simulink model "ts_b04_grid_PASS"  (R2024b)
settings: Solver=FixedStepDiscrete  StartTime=0.0  StopTime=12  FixedStep=Ts  RelTol=1e-4
PreLoadFcn:
  | Ts=50e-6;
undefined symbols (not defined in the file): D1, Delta, DiscIntNeverNeededParam
libraries: simulink x22, spsSecondOrderFilterLib x14, spsabctodq0Lib x7, spsThreePhaseVIMeasurementLib x7, spsThreePhaseSeriesRLCLoadLib x5, spsPowerPLLDrivenPositiveSequenceLib x4, spsStairGeneratorLib x4, spsThreePhaseTransformerTwoWindingsLib x3, spsDCVoltageSourceLib x3, spsThreePhaseSeriesRLCBranchLib x3, spsPWMGeneratorPulseAveragingLib x3, spsTwoLevelConverterLib x3
(part 2 of 3)

== system ts_b04_grid_PASS/Microgrid Supervisory Control/PI regulator with anti-windup q ==
  note: Anti-windup mechanism: Method of conditionnal integration
      |
      | The integration is suspended if saturation occurs and the
      | control error is of the same sign as the control signal.
      |
      | [1] L.Rundqwist, "Anti-Reset Windup for PID Controllers," Ph.D. Thesis TRFT-1033,
      | Departement of Automatic Control, Lund Institute of Technology, Lund, Sweeden, 1991.
  Error : Inport  SampleTime=Ts
  Reset : Inport  Port=2  SampleTime=Ts
  Compare To Zero : simulink/Logic and Bit Operations/Compare To Zero  relop=>  OutDataTypeStr=uint8  ZeroCross=off
  Compare To Zero1 : simulink/Logic and Bit Operations/Compare To Zero  relop=<  OutDataTypeStr=uint8  ZeroCross=off
  Constant : Constant  Value=0
  Constant1 : Constant  Value=UpperLimit
  Constant3 : Constant  Value=LowerLimit
  Discrete-Time Integrator : DiscreteIntegrator  IntegratorMethod=Integration: Trapezoidal  ExternalReset=level  InitialCondition=Init  SampleTime=Ts  LimitOutput=on  UpperSaturationLimit=UpperLimit  LowerSaturationLimit=LowerLimit  ShowStatePort=on  ICPrevOutput=DiscIntNeverNeededParam  ICPrevScaledInput=DiscIntNeverNeededParam
  Kp4 : Gain  Gain=Kp  SaturateOnIntegerOverflow=on  SampleTime=Ts  OutDataTypeStr=Inherit: Same as input  ParamDataTypeStr=Inherit: Same as input
  Kp5 : Gain  Gain=Ki  SaturateOnIntegerOverflow=on  SampleTime=Ts  OutDataTypeStr=Inherit: Same as input  ParamDataTypeStr=Inherit: Same as input
  Logical Operator : Logic  AllPortsSameDT=off  OutDataTypeStr=boolean
  Logical Operator1 : Logic  AllPortsSameDT=off  OutDataTypeStr=boolean
  Logical Operator2 : Logic  Operator=OR  AllPortsSameDT=off  OutDataTypeStr=boolean
  Relational Operator : RelationalOperator  OutDataTypeStr=boolean  InputSameDT=off
  Relational Operator1 : RelationalOperator  Operator=<=  OutDataTypeStr=boolean  InputSameDT=off
  Saturation2 : Saturate  UpperLimit=UpperLimit  LowerLimit=LowerLimit  SampleTime=Ts
  Sum1 : Sum  InputSameDT=on  SaturateOnIntegerOverflow=on  SampleTime=Ts  OutDataTypeStr=Inherit: Same as first input
  Sum6 : Sum  InputSameDT=on  SaturateOnIntegerOverflow=on  SampleTime=Ts  OutDataTypeStr=Inherit: Same as first input
  Switch : Switch  Criteria=u2 > Threshold  SaturateOnIntegerOverflow=off  InputSameDT=off
  Zero-Order Hold : ZeroOrderHold  SampleTime=Ts
  Out : Outport  SampleTime=Ts  InitialOutput=0  VectorParamsAs1DForOutWhenUnconnected=off
  wires:
  Reset/1 -> Discrete-Time Integrator/2
  Constant/1 -> Switch/1
  Zero-Order Hold/1 -> Sum1/2, Sum6/1
  Discrete-Time Integrator/State -> Sum1/1
  Sum1/1 -> Relational Operator1/1, Relational Operator/1
  Logical Operator2/1 -> Switch/2
  Relational Operator/1 -> Logical Operator/1  "UpperLimit_is_Reached"
  Relational Operator1/1 -> Logical Operator1/1  "LowerLimit_Is_Reached"
  Constant1/1 -> Relational Operator/2
  Constant3/1 -> Relational Operator1/2
  Compare To Zero/1 -> Logical Operator/2  "Error_is_positive"
  Logical Operator/1 -> Logical Operator2/1
  Logical Operator1/1 -> Logical Operator2/2
  Compare To Zero1/1 -> Logical Operator1/2  "Error_is_negative"
  Error/1 -> Compare To Zero1/1, Compare To Zero/1, Kp4/1, Kp5/1
  Sum6/1 -> Saturation2/1
  Kp4/1 -> Zero-Order Hold/1
  Discrete-Time Integrator/1 -> Sum6/2
  Saturation2/1 -> Out/1
  Switch/1 -> Discrete-Time Integrator/1
  Kp5/1 -> Switch/3

== system ts_b04_grid_PASS/Microgrid Supervisory Control/PI regulator with anti-windup q1 ==
  note: Anti-windup mechanism: Method of conditionnal integration
      |
      | The integration is suspended if saturation occurs and the
      | control error is of the same sign as the control signal.
      |
      | [1] L.Rundqwist, "Anti-Reset Windup for PID Controllers," Ph.D. Thesis TRFT-1033,
      | Departement of Automatic Control, Lund Institute of Technology, Lund, Sweeden, 1991.
  Error : Inport  SampleTime=Ts
  Reset : Inport  Port=2  SampleTime=Ts
  Compare To Zero : simulink/Logic and Bit Operations/Compare To Zero  relop=>  OutDataTypeStr=uint8  ZeroCross=off
  Compare To Zero1 : simulink/Logic and Bit Operations/Compare To Zero  relop=<  OutDataTypeStr=uint8  ZeroCross=off
  Constant : Constant  Value=0
  Constant1 : Constant  Value=UpperLimit
  Constant3 : Constant  Value=LowerLimit
  Discrete-Time Integrator : DiscreteIntegrator  IntegratorMethod=Integration: Trapezoidal  ExternalReset=level  InitialCondition=Init  SampleTime=Ts  LimitOutput=on  UpperSaturationLimit=UpperLimit  LowerSaturationLimit=LowerLimit  ShowStatePort=on  ICPrevOutput=DiscIntNeverNeededParam  ICPrevScaledInput=DiscIntNeverNeededParam
  Kp4 : Gain  Gain=Kp  SaturateOnIntegerOverflow=on  SampleTime=Ts  OutDataTypeStr=Inherit: Same as input  ParamDataTypeStr=Inherit: Same as input
  Kp5 : Gain  Gain=Ki  SaturateOnIntegerOverflow=on  SampleTime=Ts  OutDataTypeStr=Inherit: Same as input  ParamDataTypeStr=Inherit: Same as input
  Logical Operator : Logic  AllPortsSameDT=off  OutDataTypeStr=boolean
  Logical Operator1 : Logic  AllPortsSameDT=off  OutDataTypeStr=boolean
  Logical Operator2 : Logic  Operator=OR  AllPortsSameDT=off  OutDataTypeStr=boolean
  Relational Operator : RelationalOperator  OutDataTypeStr=boolean  InputSameDT=off
  Relational Operator1 : RelationalOperator  Operator=<=  OutDataTypeStr=boolean  InputSameDT=off
  Saturation2 : Saturate  UpperLimit=UpperLimit  LowerLimit=LowerLimit  SampleTime=Ts
  Sum1 : Sum  InputSameDT=on  SaturateOnIntegerOverflow=on  SampleTime=Ts  OutDataTypeStr=Inherit: Same as first input
  Sum6 : Sum  InputSameDT=on  SaturateOnIntegerOverflow=on  SampleTime=Ts  OutDataTypeStr=Inherit: Same as first input
  Switch : Switch  Criteria=u2 > Threshold  SaturateOnIntegerOverflow=off  InputSameDT=off
  Zero-Order Hold : ZeroOrderHold  SampleTime=Ts
  Out : Outport  SampleTime=Ts  InitialOutput=0  VectorParamsAs1DForOutWhenUnconnected=off
  wires:
  Kp5/1 -> Switch/3
  Switch/1 -> Discrete-Time Integrator/1
  Saturation2/1 -> Out/1
  Discrete-Time Integrator/1 -> Sum6/2
  Kp4/1 -> Zero-Order Hold/1
  Sum6/1 -> Saturation2/1
  Error/1 -> Kp5/1, Kp4/1, Compare To Zero/1, Compare To Zero1/1
  Compare To Zero1/1 -> Logical Operator1/2  "Error_is_negative"
  Logical Operator1/1 -> Logical Operator2/2
  Logical Operator/1 -> Logical Operator2/1
  Compare To Zero/1 -> Logical Operator/2  "Error_is_positive"
  Constant3/1 -> Relational Operator1/2
  Constant1/1 -> Relational Operator/2
  Relational Operator1/1 -> Logical Operator1/1  "LowerLimit_Is_Reached"
  Relational Operator/1 -> Logical Operator/1  "UpperLimit_is_Reached"
  Logical Operator2/1 -> Switch/2
  Sum1/1 -> Relational Operator/1, Relational Operator1/1
  Discrete-Time Integrator/State -> Sum1/1
  Zero-Order Hold/1 -> Sum6/1, Sum1/2
  Constant/1 -> Switch/1
  Reset/1 -> Discrete-Time Integrator/2

== system ts_b04_grid_PASS/Inverter 1 500 kW/Control System/Current Regulator ==
  note: For Ltot >> Rtot :
  note: (Vq_prim - Vq_conv) ~ = - Id * Ltot
  note: (Vd_prim - Vd_conv) ~= + Iq * Ltot
  note: Ltot = Lxfo + Lchoke
      | Rtot = Rxfo + Rchoke
  note: Id positive --> The converter generates active power ("Inverter mode") = Active Power P positive
  note: Iq positive --> The converter absorbs reactive power ("Inductive mode") = Reactive Power Q negative
  note: Sign Convention: Current going out of the converter = positive current
  note: Current Regulator
      | (with feedforward)
  note: Vq_meas + Id*L + Iq*R + deriv(Iq)*L/wbase= Vq_conv
  note: Vd_meas + Id*R - Iq*L + deriv(Id)*L/wbase= Vd_conv
  note: harmonic filter neglected
  VdVq_meas : Inport  PortDimensions=2
  IdIq_meas : Inport  Port=2  PortDimensions=2
  IdIq_ref : Inport  Port=3  PortDimensions=2
  Add1 : Sum  Inputs=++-
  Add2 : Sum
  Add3 : Sum  Inputs=+++
  Demux : Demux  Outputs=2
  Demux1 : Demux  Outputs=2
  Ltot_pu1 : Gain  Gain=Lff  SaturateOnIntegerOverflow=on  OutDataTypeStr=Inherit: Same as input  ParamDataTypeStr=Inherit: Same as input
  Ltot_pu2 : Gain  Gain=Lff  SaturateOnIntegerOverflow=on  OutDataTypeStr=Inherit: Same as input  ParamDataTypeStr=Inherit: Same as input
  Mux : Mux  Inputs=2
  PI regulator with anti-windup D : Subsystem  DialogController=POWERSYS.PowerSysDialog  mask(Discrete PI Controller){Kp=Kp_Ireg, Ki=Ki_Ireg, Par_Limits=Limits_Ireg, Init=0, Ts=Ts}
      mask prompts: Kp "Proportional gain (Kp):"; Ki "Integral gain (Ki):"; Par_Limits "Output limits: [ Upper   Lower ]"; Init "Output initial value:"; Ts "Sample time:"
      mask help: This block implements a discrete PI controller.
      mask init:
      | UpperLimit=Par_Limits(1);
      | LowerLimit=Par_Limits(2);
      | power_initmask();
      mask Help: This block is part of a subset of blocks in the Extras library that does not have documentation associated with it, other than the block mask description.
      mask Display: disp('PI');
  Rtot_pu1 : Gain  Gain=Rff  SaturateOnIntegerOverflow=on  OutDataTypeStr=Inherit: Same as input  ParamDataTypeStr=Inherit: Same as input
  Rtot_pu5 : Gain  Gain=Rff  SaturateOnIntegerOverflow=on  OutDataTypeStr=Inherit: Same as input  ParamDataTypeStr=Inherit: Same as input
  Saturation : Saturate  UpperLimit=Limits_Ireg(1)  LowerLimit=Limits_Ireg(2)
  Sum : Sum  Inputs=|-+
  VdVq_conv : Outport  VectorParamsAs1DForOutWhenUnconnected=off
  PIdq : Outport  Port=2  VectorParamsAs1DForOutWhenUnconnected=off
  wires:
  Add3/1 -> Mux/2
  Demux/2 -> Add3/1
  Add1/1 -> Mux/1  "Feedforward"
  Ltot_pu2/1 -> Add3/3
  Rtot_pu5/1 -> Add3/2
  Demux1/2 -> Rtot_pu5/1, Ltot_pu1/1
  Ltot_pu1/1 -> Add1/3
  Demux1/1 -> Ltot_pu2/1, Rtot_pu1/1
  Rtot_pu1/1 -> Add1/2
  Demux/1 -> Add1/1
  VdVq_meas/1 -> Demux/1
  Saturation/1 -> VdVq_conv/1
  Add2/1 -> Saturation/1
  IdIq_meas/1 -> Sum/1
  IdIq_ref/1 -> Demux1/1, Sum/2
  Sum/1 -> PI regulator with anti-windup D/1(Error)
  PI regulator with anti-windup D/1(Out) -> Add2/1, PIdq/1  "PI"
  Mux/1 -> Add2/2

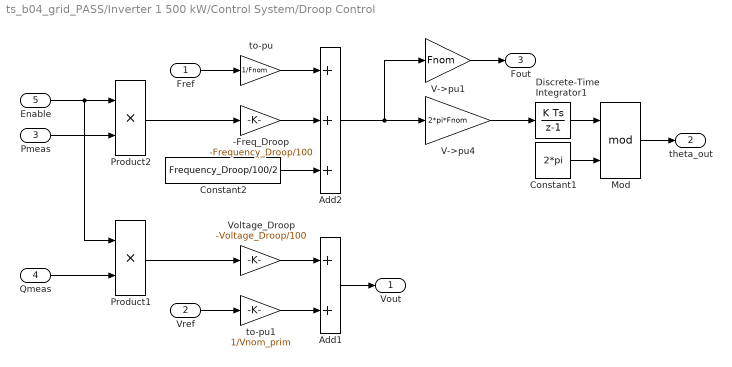
== system ts_b04_grid_PASS/Inverter 1 500 kW/Control System/Droop Control ==
  Fref : Inport  PortDimensions=1
  Vref : Inport  Port=2  PortDimensions=1
  Pmeas : Inport  Port=3
  Qmeas : Inport  Port=4
  Enable : Inport  Port=5
  -Freq_Droop : Gain  Gain=-Frequency_Droop/100
  Add1 : Sum
  Add2 : Sum  Inputs=+++
  Constant1 : Constant  Value=2*pi
  Constant2 : Constant  Value=Frequency_Droop/100/2
  Discrete-Time Integrator1 : DiscreteIntegrator  SampleTime=Ts  ICPrevOutput=DiscIntNeverNeededParam  ICPrevScaledInput=DiscIntNeverNeededParam
  Mod : Math  Operator=mod
  Product1 : Product
  Product2 : Product
  V->pu1 : Gain  Gain=Fnom  SaturateOnIntegerOverflow=on  OutDataTypeStr=Inherit: Same as input  ParamDataTypeStr=Inherit: Same as input
  V->pu4 : Gain  Gain=2*pi*Fnom  SaturateOnIntegerOverflow=on  OutDataTypeStr=Inherit: Same as input  ParamDataTypeStr=Inherit: Same as input
  Voltage_Droop : Gain  Gain=-Voltage_Droop/100
  to-pu : Gain  Gain=1/Fnom
  to-pu1 : Gain  Gain=1/Vnom_prim
  Vout : Outport
  theta_out : Outport  Port=2
  Fout : Outport  Port=3
  wires:
  Constant1/1 -> Mod/2
  -Freq_Droop/1 -> Add2/2
  Discrete-Time Integrator1/1 -> Mod/1
  Add2/1 -> V->pu4/1, V->pu1/1
  Enable/1 -> Product1/1, Product2/1
  Pmeas/1 -> Product2/2
  to-pu/1 -> Add2/1
  V->pu4/1 -> Discrete-Time Integrator1/1
  Fref/1 -> to-pu/1
  Vref/1 -> to-pu1/1
  to-pu1/1 -> Add1/2
  Add1/1 -> Vout/1
  Mod/1 -> theta_out/1
  Voltage_Droop/1 -> Add1/1
  Qmeas/1 -> Product1/2
  Product2/1 -> -Freq_Droop/1
  Product1/1 -> Voltage_Droop/1
  Constant2/1 -> Add2/3
  V->pu1/1 -> Fout/1

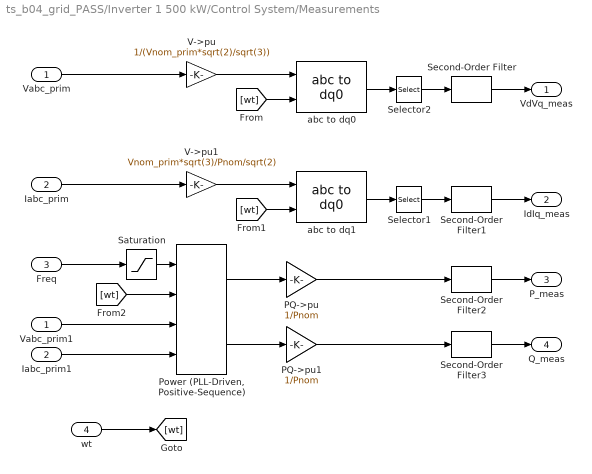
== system ts_b04_grid_PASS/Inverter 1 500 kW/Control System/Measurements ==
  Vabc_prim : Inport
  Iabc_prim : Inport  Port=2
  Freq : Inport  Port=3
  wt : Inport  Port=4
  Iabc_prim1 : InportShadow  Port=2
  PQ->pu : Gain  Gain=1/Pnom  SaturateOnIntegerOverflow=on  OutDataTypeStr=Inherit: Same as input  ParamDataTypeStr=Inherit: Same as input
  PQ->pu1 : Gain  Gain=1/Pnom  SaturateOnIntegerOverflow=on  OutDataTypeStr=Inherit: Same as input  ParamDataTypeStr=Inherit: Same as input
  "Power (PLL-Driven, Positive-Sequence)" : spsPowerPLLDrivenPositiveSequenceLib/Power (PLL-Driven, Positive-Sequence)  Finit=50  Fmin=45  Vinit=[1, 0]  Iinit=[1, 0]  Ts=Ts
  Saturation : Saturate  UpperLimit=55  LowerLimit=45
  Second-Order Filter{,1..3} (4 alike) : spsSecondOrderFilterLib/Second-Order Filter  FilterType=Lowpass  Fo=fn_Filter  Zeta=1  Ts=Ts  Initialize=off  Vac_Init=[0, 0, 50]  Vdc_Init=0  PlotResponse=off  FreqRange=[0, 500, 1]
  Selector1 : Selector  InputPortWidth=3  IndexOptions=Index vector (dialog)  Indices=[1 2]  OutputSizes=1
  Selector2 : Selector  InputPortWidth=3  IndexOptions=Index vector (dialog)  Indices=[1 2]  OutputSizes=1
  V->pu : Gain  Gain=1/(Vnom_prim*sqrt(2)/sqrt(3))  SaturateOnIntegerOverflow=on  OutDataTypeStr=Inherit: Same as input  ParamDataTypeStr=Inherit: Same as input
  V->pu1 : Gain  Gain=Vnom_prim*sqrt(3)/Pnom/sqrt(2)  SaturateOnIntegerOverflow=on  OutDataTypeStr=Inherit: Same as input  ParamDataTypeStr=Inherit: Same as input
  Vabc_prim1 : InportShadow
  abc to dq0 : spsabctodq0Lib/abc to dq0  Alignment=90 degrees behind phase A axis
  abc to dq1 : spsabctodq0Lib/abc to dq0  Alignment=90 degrees behind phase A axis
  VdVq_meas : Outport  VectorParamsAs1DForOutWhenUnconnected=off
  IdIq_meas : Outport  Port=2  VectorParamsAs1DForOutWhenUnconnected=off
  P_meas : Outport  Port=3  VectorParamsAs1DForOutWhenUnconnected=off
  Q_meas : Outport  Port=4  VectorParamsAs1DForOutWhenUnconnected=off
  wires:
  Iabc_prim1/1 -> "Power (PLL-Driven, Positive-Sequence)"/4
  Vabc_prim1/1 -> "Power (PLL-Driven, Positive-Sequence)"/3
  abc to dq0/1 -> Selector2/1
  Iabc_prim/1 -> V->pu1/1
  Vabc_prim/1 -> V->pu/1
  abc to dq1/1 -> Selector1/1
  V->pu/1 -> abc to dq0/1
  V->pu1/1 -> abc to dq1/1
  Freq/1 -> Saturation/1
  Selector2/1 -> Second-Order Filter/1
  Selector1/1 -> Second-Order Filter1/1
  Second-Order Filter/1 -> VdVq_meas/1
  Second-Order Filter1/1 -> IdIq_meas/1
  [wt] -> abc to dq0/2
  [wt] -> abc to dq1/2
  [wt] -> "Power (PLL-Driven, Positive-Sequence)"/2
  "Power (PLL-Driven, Positive-Sequence)"/1 -> PQ->pu/1
  Second-Order Filter2/1 -> P_meas/1
  PQ->pu1/1 -> Second-Order Filter3/1
  Second-Order Filter3/1 -> Q_meas/1
  PQ->pu/1 -> Second-Order Filter2/1
  "Power (PLL-Driven, Positive-Sequence)"/2 -> PQ->pu1/1
  wt/1 -> [wt]
  Saturation/1 -> "Power (PLL-Driven, Positive-Sequence)"/1

== system ts_b04_grid_PASS/Inverter 1 500 kW/Control System/Voltage Regulators ==
  note: Iqref limit set 0.5 pu
  Vq : Inport  PortDimensions=1
  Vq_ref : Inport  Port=2  PortDimensions=1
  On : Inport  Port=3  PortDimensions=1
  Vd : Inport  Port=4  PortDimensions=1
  Vd_ref : Inport  Port=5  PortDimensions=1
  Constant1 : Constant  Value=0
  Constant2 : Constant
  Mux : Mux  Inputs=2
  PI regulator with anti-windup 1 : Subsystem  DialogController=POWERSYS.PowerSysDialog  mask(Discrete PI Controller){Kp=Kp_Vreg, Ki=Ki_Vreg, Par_Limits=[0.5, -0.5], Init=0, Ts=Ts}
      mask prompts: Kp "Proportional gain (Kp):"; Ki "Integral gain (Ki):"; Par_Limits "Output limits: [ Upper   Lower ]"; Init "Output initial value:"; Ts "Sample time:"
      mask help: This block implements a discrete PI controller.
      mask init:
      | UpperLimit=Par_Limits(1);
      | LowerLimit=Par_Limits(2);
      | power_initmask();
      mask Help: This block is part of a subset of blocks in the Extras library that does not have documentation associated with it, other than the block mask description.
      mask Display: disp('PI');
  PI regulator with anti-windup 2 : Subsystem  DialogController=POWERSYS.PowerSysDialog  mask(Discrete PI Controller){Kp=Kp_Vreg, Ki=Ki_Vreg, Par_Limits=Limits_Vreg, Init=0, Ts=Ts}
      mask prompts: Kp "Proportional gain (Kp):"; Ki "Integral gain (Ki):"; Par_Limits "Output limits: [ Upper   Lower ]"; Init "Output initial value:"; Ts "Sample time:"
      mask help: This block implements a discrete PI controller.
      mask init:
      | UpperLimit=Par_Limits(1);
      | LowerLimit=Par_Limits(2);
      | power_initmask();
      mask Help: This block is part of a subset of blocks in the Extras library that does not have documentation associated with it, other than the block mask description.
      mask Display: disp('PI');
  Sum : Sum  Inputs=|+-
  Sum1 : Sum  Inputs=|+-
  Switch : Switch  Criteria=u2 ~= 0  SaturateOnIntegerOverflow=off  InputSameDT=off
  IdIq_ref : Outport  InitialOutput=0  VectorParamsAs1DForOutWhenUnconnected=off
  wires:
  Constant1/1 -> Switch/1
  On/1 -> Switch/2
  Switch/1 -> PI regulator with anti-windup 2/2(Reset), PI regulator with anti-windup 1/2(Reset)
  Constant2/1 -> Switch/3
  Vq_ref/1 -> Sum/1
  Vq/1 -> Sum/2
  Sum/1 -> PI regulator with anti-windup 1/1(Error)
  Sum1/1 -> PI regulator with anti-windup 2/1(Error)
  Vd/1 -> Sum1/1
  Vd_ref/1 -> Sum1/2
  PI regulator with anti-windup 2/1(Out) -> Mux/2
  Mux/1 -> IdIq_ref/1
  PI regulator with anti-windup 1/1(Out) -> Mux/1

== system ts_b04_grid_PASS/Inverter 1 500 kW/Control System/Vref Generation ==
  note: (Correction for delai of Ts)
  note: (Correction for transformer
      |  D1 connection)
  wt : Inport
  VdVq_conv : Inport  Port=2
  Vdc_meas : Inport  Port=3
  Add1 : Sum  Inputs=++++
  Add2 : Sum
  Complex to Magnitude-Angle : ComplexToMagnitudeAngle
  Constant : Constant  Value=-pi/6
  Constant2 : Constant  Value="[ 0  -2*pi/3  2*pi/3  ]"
  Constant3 : Constant  Value=Vnom_sec*sqrt(2)/sqrt(3)
  Constant4 : Constant  Value=Ts*Fnom*(2*pi)
  Demux1 : Demux  Outputs=2
  Gain1 : Gain  Gain=1/2
  Product : Product  Inputs=*/  RndMeth=Zero
  Product1 : Product  Inputs=*/  RndMeth=Zero
  Product2 : Product  Inputs=**  RndMeth=Zero
  Real-Imag to Complex : RealImagToComplex
  Saturation : Saturate  UpperLimit=1  LowerLimit=0
  Trigonometric Function : Trigonometry
  Vref : Outport  VectorParamsAs1DForOutWhenUnconnected=off
  ModIndex : Outport  Port=2  VectorParamsAs1DForOutWhenUnconnected=off
  wires:
  Constant4/1 -> Add1/4
  wt/1 -> Add1/1
  Product2/1 -> Vref/1
  Trigonometric Function/1 -> Product2/2
  Saturation/1 -> ModIndex/1, Product2/1
  Add2/1 -> Trigonometric Function/1
  Add1/1 -> Add2/2
  Complex to Magnitude-Angle/2 -> Add2/1
  Product/1 -> Product1/2
  Constant3/1 -> Product/2
  Constant/1 -> Add1/3
  Constant2/1 -> Add1/2
  Demux1/2 -> Real-Imag to Complex/2
  Demux1/1 -> Real-Imag to Complex/1
  Real-Imag to Complex/1 -> Complex to Magnitude-Angle/1
  Gain1/1 -> Product/1
  Product1/1 -> Demux1/1
  VdVq_conv/1 -> Product1/1
  Vdc_meas/1 -> Gain1/1
  Complex to Magnitude-Angle/1 -> Saturation/1

== system ts_b04_grid_PASS/Inverter 2 300 kW/Control System/Current Regulator ==
  note: For Ltot >> Rtot :
  note: (Vq_prim - Vq_conv) ~ = - Id * Ltot
  note: (Vd_prim - Vd_conv) ~= + Iq * Ltot
  note: Ltot = Lxfo + Lchoke
      | Rtot = Rxfo + Rchoke
  note: Id positive --> The converter generates active power ("Inverter mode") = Active Power P positive
  note: Iq positive --> The converter absorbs reactive power ("Inductive mode") = Reactive Power Q negative
  note: Sign Convention: Current going out of the converter = positive current
  note: Current Regulator
      | (with feedforward)
  note: Vq_meas + Id*L + Iq*R + deriv(Iq)*L/wbase= Vq_conv
  note: Vd_meas + Id*R - Iq*L + deriv(Id)*L/wbase= Vd_conv
  note: harmonic filter neglected
  VdVq_meas : Inport  PortDimensions=2
  IdIq_meas : Inport  Port=2  PortDimensions=2
  IdIq_ref : Inport  Port=3  PortDimensions=2
  Add1 : Sum  Inputs=++-
  Add2 : Sum
  Add3 : Sum  Inputs=+++
  Demux : Demux  Outputs=2
  Demux1 : Demux  Outputs=2
  Ltot_pu1 : Gain  Gain=Lff  SaturateOnIntegerOverflow=on  OutDataTypeStr=Inherit: Same as input  ParamDataTypeStr=Inherit: Same as input
  Ltot_pu2 : Gain  Gain=Lff  SaturateOnIntegerOverflow=on  OutDataTypeStr=Inherit: Same as input  ParamDataTypeStr=Inherit: Same as input
  Mux : Mux  Inputs=2
  PI regulator with anti-windup D : Subsystem  DialogController=POWERSYS.PowerSysDialog  mask(Discrete PI Controller){Kp=Kp_Ireg, Ki=Ki_Ireg, Par_Limits=Limits_Ireg, Init=0, Ts=Ts}
      mask prompts: Kp "Proportional gain (Kp):"; Ki "Integral gain (Ki):"; Par_Limits "Output limits: [ Upper   Lower ]"; Init "Output initial value:"; Ts "Sample time:"
      mask help: This block implements a discrete PI controller.
      mask init:
      | UpperLimit=Par_Limits(1);
      | LowerLimit=Par_Limits(2);
      | power_initmask();
      mask Help: This block is part of a subset of blocks in the Extras library that does not have documentation associated with it, other than the block mask description.
      mask Display: disp('PI');
  Rtot_pu1 : Gain  Gain=Rff  SaturateOnIntegerOverflow=on  OutDataTypeStr=Inherit: Same as input  ParamDataTypeStr=Inherit: Same as input
  Rtot_pu5 : Gain  Gain=Rff  SaturateOnIntegerOverflow=on  OutDataTypeStr=Inherit: Same as input  ParamDataTypeStr=Inherit: Same as input
  Saturation : Saturate  UpperLimit=Limits_Ireg(1)  LowerLimit=Limits_Ireg(2)
  Sum : Sum  Inputs=|-+
  VdVq_conv : Outport  VectorParamsAs1DForOutWhenUnconnected=off
  PIdq : Outport  Port=2  VectorParamsAs1DForOutWhenUnconnected=off
  wires:
  Add3/1 -> Mux/2
  Demux/2 -> Add3/1
  Add1/1 -> Mux/1  "Feedforward"
  Ltot_pu2/1 -> Add3/3
  Rtot_pu5/1 -> Add3/2
  Demux1/2 -> Rtot_pu5/1, Ltot_pu1/1
  Ltot_pu1/1 -> Add1/3
  Demux1/1 -> Ltot_pu2/1, Rtot_pu1/1
  Rtot_pu1/1 -> Add1/2
  Demux/1 -> Add1/1
  VdVq_meas/1 -> Demux/1
  Saturation/1 -> VdVq_conv/1
  Add2/1 -> Saturation/1
  IdIq_meas/1 -> Sum/1
  IdIq_ref/1 -> Demux1/1, Sum/2
  Sum/1 -> PI regulator with anti-windup D/1(Error)
  PI regulator with anti-windup D/1(Out) -> Add2/1, PIdq/1  "PI"
  Mux/1 -> Add2/2

== system ts_b04_grid_PASS/Inverter 2 300 kW/Control System/Droop Control ==
  Fref : Inport  PortDimensions=1
  Vref : Inport  Port=2  PortDimensions=1
  Pmeas : Inport  Port=3
  Qmeas : Inport  Port=4
  Enable : Inport  Port=5
  -Freq_Droop : Gain  Gain=-Frequency_Droop/100
  Add1 : Sum
  Add2 : Sum  Inputs=+++
  Constant1 : Constant  Value=2*pi
  Constant2 : Constant  Value=Frequency_Droop/100/2
  Discrete-Time Integrator1 : DiscreteIntegrator  SampleTime=Ts  ICPrevOutput=DiscIntNeverNeededParam  ICPrevScaledInput=DiscIntNeverNeededParam
  Mod : Math  Operator=mod
  Product1 : Product
  Product2 : Product
  V->pu1 : Gain  Gain=Fnom  SaturateOnIntegerOverflow=on  OutDataTypeStr=Inherit: Same as input  ParamDataTypeStr=Inherit: Same as input
  V->pu4 : Gain  Gain=2*pi*Fnom  SaturateOnIntegerOverflow=on  OutDataTypeStr=Inherit: Same as input  ParamDataTypeStr=Inherit: Same as input
  Voltage_Droop : Gain  Gain=-Voltage_Droop/100
  to-pu : Gain  Gain=1/Fnom
  to-pu1 : Gain  Gain=1/Vnom_prim
  Vout : Outport
  theta_out : Outport  Port=2
  Fout : Outport  Port=3
  wires:
  Constant1/1 -> Mod/2
  -Freq_Droop/1 -> Add2/2
  Discrete-Time Integrator1/1 -> Mod/1
  Add2/1 -> V->pu4/1, V->pu1/1
  Enable/1 -> Product1/1, Product2/1
  Pmeas/1 -> Product2/2
  to-pu/1 -> Add2/1
  V->pu4/1 -> Discrete-Time Integrator1/1
  Fref/1 -> to-pu/1
  Vref/1 -> to-pu1/1
  to-pu1/1 -> Add1/2
  Add1/1 -> Vout/1
  Mod/1 -> theta_out/1
  Voltage_Droop/1 -> Add1/1
  Qmeas/1 -> Product1/2
  Product2/1 -> -Freq_Droop/1
  Product1/1 -> Voltage_Droop/1
  Constant2/1 -> Add2/3
  V->pu1/1 -> Fout/1

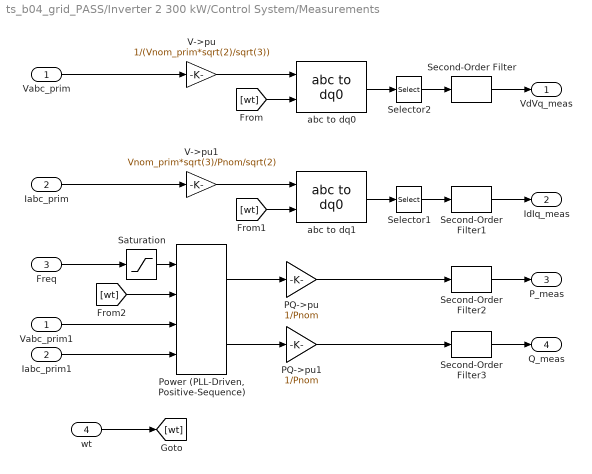
== system ts_b04_grid_PASS/Inverter 2 300 kW/Control System/Measurements ==
  Vabc_prim : Inport
  Iabc_prim : Inport  Port=2
  Freq : Inport  Port=3
  wt : Inport  Port=4
  Iabc_prim1 : InportShadow  Port=2
  PQ->pu : Gain  Gain=1/Pnom  SaturateOnIntegerOverflow=on  OutDataTypeStr=Inherit: Same as input  ParamDataTypeStr=Inherit: Same as input
  PQ->pu1 : Gain  Gain=1/Pnom  SaturateOnIntegerOverflow=on  OutDataTypeStr=Inherit: Same as input  ParamDataTypeStr=Inherit: Same as input
  "Power (PLL-Driven, Positive-Sequence)" : spsPowerPLLDrivenPositiveSequenceLib/Power (PLL-Driven, Positive-Sequence)  Finit=50  Fmin=45  Vinit=[1, 0]  Iinit=[1, 0]  Ts=Ts
  Saturation : Saturate  UpperLimit=55  LowerLimit=45
  Second-Order Filter{,1..3} (4 alike) : spsSecondOrderFilterLib/Second-Order Filter  FilterType=Lowpass  Fo=fn_Filter  Zeta=1  Ts=Ts  Initialize=off  Vac_Init=[0, 0, 50]  Vdc_Init=0  PlotResponse=off  FreqRange=[0, 500, 1]
  Selector1 : Selector  InputPortWidth=3  IndexOptions=Index vector (dialog)  Indices=[1 2]  OutputSizes=1
  Selector2 : Selector  InputPortWidth=3  IndexOptions=Index vector (dialog)  Indices=[1 2]  OutputSizes=1
  V->pu : Gain  Gain=1/(Vnom_prim*sqrt(2)/sqrt(3))  SaturateOnIntegerOverflow=on  OutDataTypeStr=Inherit: Same as input  ParamDataTypeStr=Inherit: Same as input
  V->pu1 : Gain  Gain=Vnom_prim*sqrt(3)/Pnom/sqrt(2)  SaturateOnIntegerOverflow=on  OutDataTypeStr=Inherit: Same as input  ParamDataTypeStr=Inherit: Same as input
  Vabc_prim1 : InportShadow
  abc to dq0 : spsabctodq0Lib/abc to dq0  Alignment=90 degrees behind phase A axis
  abc to dq1 : spsabctodq0Lib/abc to dq0  Alignment=90 degrees behind phase A axis
  VdVq_meas : Outport  VectorParamsAs1DForOutWhenUnconnected=off
  IdIq_meas : Outport  Port=2  VectorParamsAs1DForOutWhenUnconnected=off
  P_meas : Outport  Port=3  VectorParamsAs1DForOutWhenUnconnected=off
  Q_meas : Outport  Port=4  VectorParamsAs1DForOutWhenUnconnected=off
  wires:
  Iabc_prim1/1 -> "Power (PLL-Driven, Positive-Sequence)"/4
  Vabc_prim1/1 -> "Power (PLL-Driven, Positive-Sequence)"/3
  abc to dq0/1 -> Selector2/1
  Iabc_prim/1 -> V->pu1/1
  Vabc_prim/1 -> V->pu/1
  abc to dq1/1 -> Selector1/1
  V->pu/1 -> abc to dq0/1
  V->pu1/1 -> abc to dq1/1
  Freq/1 -> Saturation/1
  Selector2/1 -> Second-Order Filter/1
  Selector1/1 -> Second-Order Filter1/1
  Second-Order Filter/1 -> VdVq_meas/1
  Second-Order Filter1/1 -> IdIq_meas/1
  [wt] -> abc to dq0/2
  [wt] -> abc to dq1/2
  [wt] -> "Power (PLL-Driven, Positive-Sequence)"/2
  "Power (PLL-Driven, Positive-Sequence)"/1 -> PQ->pu/1
  Second-Order Filter2/1 -> P_meas/1
  PQ->pu1/1 -> Second-Order Filter3/1
  Second-Order Filter3/1 -> Q_meas/1
  PQ->pu/1 -> Second-Order Filter2/1
  "Power (PLL-Driven, Positive-Sequence)"/2 -> PQ->pu1/1
  wt/1 -> [wt]
  Saturation/1 -> "Power (PLL-Driven, Positive-Sequence)"/1

== system ts_b04_grid_PASS/Inverter 2 300 kW/Control System/Voltage Regulators ==
  note: Iqref limit set 0.5 pu
  Vq : Inport  PortDimensions=1
  Vq_ref : Inport  Port=2  PortDimensions=1
  On : Inport  Port=3  PortDimensions=1
  Vd : Inport  Port=4  PortDimensions=1
  Vd_ref : Inport  Port=5  PortDimensions=1
  Constant1 : Constant  Value=0
  Constant2 : Constant
  Mux : Mux  Inputs=2
  PI regulator with anti-windup 1 : Subsystem  DialogController=POWERSYS.PowerSysDialog  mask(Discrete PI Controller){Kp=Kp_Vreg, Ki=Ki_Vreg, Par_Limits=[0.5, -0.5], Init=0, Ts=Ts}
      mask prompts: Kp "Proportional gain (Kp):"; Ki "Integral gain (Ki):"; Par_Limits "Output limits: [ Upper   Lower ]"; Init "Output initial value:"; Ts "Sample time:"
      mask help: This block implements a discrete PI controller.
      mask init:
      | UpperLimit=Par_Limits(1);
      | LowerLimit=Par_Limits(2);
      | power_initmask();
      mask Help: This block is part of a subset of blocks in the Extras library that does not have documentation associated with it, other than the block mask description.
      mask Display: disp('PI');
  PI regulator with anti-windup 2 : Subsystem  DialogController=POWERSYS.PowerSysDialog  mask(Discrete PI Controller){Kp=Kp_Vreg, Ki=Ki_Vreg, Par_Limits=Limits_Vreg, Init=0, Ts=Ts}
      mask prompts: Kp "Proportional gain (Kp):"; Ki "Integral gain (Ki):"; Par_Limits "Output limits: [ Upper   Lower ]"; Init "Output initial value:"; Ts "Sample time:"
      mask help: This block implements a discrete PI controller.
      mask init:
      | UpperLimit=Par_Limits(1);
      | LowerLimit=Par_Limits(2);
      | power_initmask();
      mask Help: This block is part of a subset of blocks in the Extras library that does not have documentation associated with it, other than the block mask description.
      mask Display: disp('PI');
  Sum : Sum  Inputs=|+-
  Sum1 : Sum  Inputs=|+-
  Switch : Switch  Criteria=u2 ~= 0  SaturateOnIntegerOverflow=off  InputSameDT=off
  IdIq_ref : Outport  InitialOutput=0  VectorParamsAs1DForOutWhenUnconnected=off
  wires:
  Constant1/1 -> Switch/1
  On/1 -> Switch/2
  Switch/1 -> PI regulator with anti-windup 2/2(Reset), PI regulator with anti-windup 1/2(Reset)
  Constant2/1 -> Switch/3
  Vq_ref/1 -> Sum/1
  Vq/1 -> Sum/2
  Sum/1 -> PI regulator with anti-windup 1/1(Error)
  Sum1/1 -> PI regulator with anti-windup 2/1(Error)
  Vd/1 -> Sum1/1
  Vd_ref/1 -> Sum1/2
  PI regulator with anti-windup 2/1(Out) -> Mux/2
  Mux/1 -> IdIq_ref/1
  PI regulator with anti-windup 1/1(Out) -> Mux/1

== system ts_b04_grid_PASS/Inverter 2 300 kW/Control System/Vref Generation ==
  note: (Correction for delai of Ts)
  note: (Correction for transformer
      |  D1 connection)
  wt : Inport
  VdVq_conv : Inport  Port=2
  Vdc_meas : Inport  Port=3
  Add1 : Sum  Inputs=++++
  Add2 : Sum
  Complex to Magnitude-Angle : ComplexToMagnitudeAngle
  Constant : Constant  Value=-pi/6
  Constant2 : Constant  Value="[ 0  -2*pi/3  2*pi/3  ]"
  Constant3 : Constant  Value=Vnom_sec*sqrt(2)/sqrt(3)
  Constant4 : Constant  Value=Ts*Fnom*(2*pi)
  Demux1 : Demux  Outputs=2
  Gain1 : Gain  Gain=1/2
  Product : Product  Inputs=*/  RndMeth=Zero
  Product1 : Product  Inputs=*/  RndMeth=Zero
  Product2 : Product  Inputs=**  RndMeth=Zero
  Real-Imag to Complex : RealImagToComplex
  Saturation : Saturate  UpperLimit=1  LowerLimit=0
  Trigonometric Function : Trigonometry
  Vref : Outport  VectorParamsAs1DForOutWhenUnconnected=off
  ModIndex : Outport  Port=2  VectorParamsAs1DForOutWhenUnconnected=off
  wires:
  Constant4/1 -> Add1/4
  wt/1 -> Add1/1
  Product2/1 -> Vref/1
  Trigonometric Function/1 -> Product2/2
  Saturation/1 -> ModIndex/1, Product2/1
  Add2/1 -> Trigonometric Function/1
  Add1/1 -> Add2/2
  Complex to Magnitude-Angle/2 -> Add2/1
  Product/1 -> Product1/2
  Constant3/1 -> Product/2
  Constant/1 -> Add1/3
  Constant2/1 -> Add1/2
  Demux1/2 -> Real-Imag to Complex/2
  Demux1/1 -> Real-Imag to Complex/1
  Real-Imag to Complex/1 -> Complex to Magnitude-Angle/1
  Gain1/1 -> Product/1
  Product1/1 -> Demux1/1
  VdVq_conv/1 -> Product1/1
  Vdc_meas/1 -> Gain1/1
  Complex to Magnitude-Angle/1 -> Saturation/1

== system ts_b04_grid_PASS/Inverter 3 200 kW/Control System/Current Regulator ==
  note: For Ltot >> Rtot :
  note: (Vq_prim - Vq_conv) ~ = - Id * Ltot
  note: (Vd_prim - Vd_conv) ~= + Iq * Ltot
  note: Ltot = Lxfo + Lchoke
      | Rtot = Rxfo + Rchoke
  note: Id positive --> The converter generates active power ("Inverter mode") = Active Power P positive
  note: Iq positive --> The converter absorbs reactive power ("Inductive mode") = Reactive Power Q negative
  note: Sign Convention: Current going out of the converter = positive current
  note: Current Regulator
      | (with feedforward)
  note: Vq_meas + Id*L + Iq*R + deriv(Iq)*L/wbase= Vq_conv
  note: Vd_meas + Id*R - Iq*L + deriv(Id)*L/wbase= Vd_conv
  note: harmonic filter neglected
  VdVq_meas : Inport  PortDimensions=2
  IdIq_meas : Inport  Port=2  PortDimensions=2
  IdIq_ref : Inport  Port=3  PortDimensions=2
  Add1 : Sum  Inputs=++-
  Add2 : Sum
  Add3 : Sum  Inputs=+++
  Demux : Demux  Outputs=2
  Demux1 : Demux  Outputs=2
  Ltot_pu1 : Gain  Gain=Lff  SaturateOnIntegerOverflow=on  OutDataTypeStr=Inherit: Same as input  ParamDataTypeStr=Inherit: Same as input
  Ltot_pu2 : Gain  Gain=Lff  SaturateOnIntegerOverflow=on  OutDataTypeStr=Inherit: Same as input  ParamDataTypeStr=Inherit: Same as input
  Mux : Mux  Inputs=2
  PI regulator with anti-windup D : Subsystem  DialogController=POWERSYS.PowerSysDialog  mask(Discrete PI Controller){Kp=Kp_Ireg, Ki=Ki_Ireg, Par_Limits=Limits_Ireg, Init=0, Ts=Ts}
      mask prompts: Kp "Proportional gain (Kp):"; Ki "Integral gain (Ki):"; Par_Limits "Output limits: [ Upper   Lower ]"; Init "Output initial value:"; Ts "Sample time:"
      mask help: This block implements a discrete PI controller.
      mask init:
      | UpperLimit=Par_Limits(1);
      | LowerLimit=Par_Limits(2);
      | power_initmask();
      mask Help: This block is part of a subset of blocks in the Extras library that does not have documentation associated with it, other than the block mask description.
      mask Display: disp('PI');
  Rtot_pu1 : Gain  Gain=Rff  SaturateOnIntegerOverflow=on  OutDataTypeStr=Inherit: Same as input  ParamDataTypeStr=Inherit: Same as input
  Rtot_pu5 : Gain  Gain=Rff  SaturateOnIntegerOverflow=on  OutDataTypeStr=Inherit: Same as input  ParamDataTypeStr=Inherit: Same as input
  Saturation : Saturate  UpperLimit=Limits_Ireg(1)  LowerLimit=Limits_Ireg(2)
  Sum : Sum  Inputs=|-+
  VdVq_conv : Outport  VectorParamsAs1DForOutWhenUnconnected=off
  PIdq : Outport  Port=2  VectorParamsAs1DForOutWhenUnconnected=off
  wires:
  Add3/1 -> Mux/2
  Demux/2 -> Add3/1
  Add1/1 -> Mux/1  "Feedforward"
  Ltot_pu2/1 -> Add3/3
  Rtot_pu5/1 -> Add3/2
  Demux1/2 -> Rtot_pu5/1, Ltot_pu1/1
  Ltot_pu1/1 -> Add1/3
  Demux1/1 -> Ltot_pu2/1, Rtot_pu1/1
  Rtot_pu1/1 -> Add1/2
  Demux/1 -> Add1/1
  VdVq_meas/1 -> Demux/1
  Saturation/1 -> VdVq_conv/1
  Add2/1 -> Saturation/1
  IdIq_meas/1 -> Sum/1
  IdIq_ref/1 -> Demux1/1, Sum/2
  Sum/1 -> PI regulator with anti-windup D/1(Error)
  PI regulator with anti-windup D/1(Out) -> Add2/1, PIdq/1  "PI"
  Mux/1 -> Add2/2

== system ts_b04_grid_PASS/Inverter 3 200 kW/Control System/Droop Control ==
  Fref : Inport  PortDimensions=1
  Vref : Inport  Port=2  PortDimensions=1
  Pmeas : Inport  Port=3
  Qmeas : Inport  Port=4
  Enable : Inport  Port=5
  -Freq_Droop : Gain  Gain=-Frequency_Droop/100
  Add1 : Sum
  Add2 : Sum  Inputs=+++
  Constant1 : Constant  Value=2*pi
  Constant2 : Constant  Value=Frequency_Droop/100/2
  Discrete-Time Integrator1 : DiscreteIntegrator  SampleTime=Ts  ICPrevOutput=DiscIntNeverNeededParam  ICPrevScaledInput=DiscIntNeverNeededParam
  Mod : Math  Operator=mod
  Product1 : Product
  Product2 : Product
  V->pu1 : Gain  Gain=Fnom  SaturateOnIntegerOverflow=on  OutDataTypeStr=Inherit: Same as input  ParamDataTypeStr=Inherit: Same as input
  V->pu4 : Gain  Gain=2*pi*Fnom  SaturateOnIntegerOverflow=on  OutDataTypeStr=Inherit: Same as input  ParamDataTypeStr=Inherit: Same as input
  Voltage_Droop : Gain  Gain=-Voltage_Droop/100
  to-pu : Gain  Gain=1/Fnom
  to-pu1 : Gain  Gain=1/Vnom_prim
  Vout : Outport
  theta_out : Outport  Port=2
  Fout : Outport  Port=3
  wires:
  Constant1/1 -> Mod/2
  -Freq_Droop/1 -> Add2/2
  Discrete-Time Integrator1/1 -> Mod/1
  Add2/1 -> V->pu4/1, V->pu1/1
  Enable/1 -> Product1/1, Product2/1
  Pmeas/1 -> Product2/2
  to-pu/1 -> Add2/1
  V->pu4/1 -> Discrete-Time Integrator1/1
  Fref/1 -> to-pu/1
  Vref/1 -> to-pu1/1
  to-pu1/1 -> Add1/2
  Add1/1 -> Vout/1
  Mod/1 -> theta_out/1
  Voltage_Droop/1 -> Add1/1
  Qmeas/1 -> Product1/2
  Product2/1 -> -Freq_Droop/1
  Product1/1 -> Voltage_Droop/1
  Constant2/1 -> Add2/3
  V->pu1/1 -> Fout/1

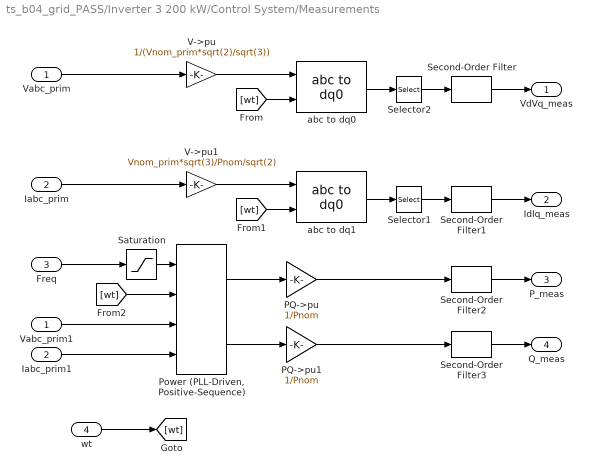
== system ts_b04_grid_PASS/Inverter 3 200 kW/Control System/Measurements ==
  Vabc_prim : Inport
  Iabc_prim : Inport  Port=2
  Freq : Inport  Port=3
  wt : Inport  Port=4
  Iabc_prim1 : InportShadow  Port=2
  PQ->pu : Gain  Gain=1/Pnom  SaturateOnIntegerOverflow=on  OutDataTypeStr=Inherit: Same as input  ParamDataTypeStr=Inherit: Same as input
  PQ->pu1 : Gain  Gain=1/Pnom  SaturateOnIntegerOverflow=on  OutDataTypeStr=Inherit: Same as input  ParamDataTypeStr=Inherit: Same as input
  "Power (PLL-Driven, Positive-Sequence)" : spsPowerPLLDrivenPositiveSequenceLib/Power (PLL-Driven, Positive-Sequence)  Finit=50  Fmin=45  Vinit=[1, 0]  Iinit=[1, 0]  Ts=Ts
  Saturation : Saturate  UpperLimit=55  LowerLimit=45
  Second-Order Filter{,1..3} (4 alike) : spsSecondOrderFilterLib/Second-Order Filter  FilterType=Lowpass  Fo=fn_Filter  Zeta=1  Ts=Ts  Initialize=off  Vac_Init=[0, 0, 50]  Vdc_Init=0  PlotResponse=off  FreqRange=[0, 500, 1]
  Selector1 : Selector  InputPortWidth=3  IndexOptions=Index vector (dialog)  Indices=[1 2]  OutputSizes=1
  Selector2 : Selector  InputPortWidth=3  IndexOptions=Index vector (dialog)  Indices=[1 2]  OutputSizes=1
  V->pu : Gain  Gain=1/(Vnom_prim*sqrt(2)/sqrt(3))  SaturateOnIntegerOverflow=on  OutDataTypeStr=Inherit: Same as input  ParamDataTypeStr=Inherit: Same as input
  V->pu1 : Gain  Gain=Vnom_prim*sqrt(3)/Pnom/sqrt(2)  SaturateOnIntegerOverflow=on  OutDataTypeStr=Inherit: Same as input  ParamDataTypeStr=Inherit: Same as input
  Vabc_prim1 : InportShadow
  abc to dq0 : spsabctodq0Lib/abc to dq0  Alignment=90 degrees behind phase A axis
  abc to dq1 : spsabctodq0Lib/abc to dq0  Alignment=90 degrees behind phase A axis
  VdVq_meas : Outport  VectorParamsAs1DForOutWhenUnconnected=off
  IdIq_meas : Outport  Port=2  VectorParamsAs1DForOutWhenUnconnected=off
  P_meas : Outport  Port=3  VectorParamsAs1DForOutWhenUnconnected=off
  Q_meas : Outport  Port=4  VectorParamsAs1DForOutWhenUnconnected=off
  wires:
  Iabc_prim1/1 -> "Power (PLL-Driven, Positive-Sequence)"/4
  Vabc_prim1/1 -> "Power (PLL-Driven, Positive-Sequence)"/3
  abc to dq0/1 -> Selector2/1
  Iabc_prim/1 -> V->pu1/1
  Vabc_prim/1 -> V->pu/1
  abc to dq1/1 -> Selector1/1
  V->pu/1 -> abc to dq0/1
  V->pu1/1 -> abc to dq1/1
  Freq/1 -> Saturation/1
  Selector2/1 -> Second-Order Filter/1
  Selector1/1 -> Second-Order Filter1/1
  Second-Order Filter/1 -> VdVq_meas/1
  Second-Order Filter1/1 -> IdIq_meas/1
  [wt] -> abc to dq0/2
  [wt] -> abc to dq1/2
  [wt] -> "Power (PLL-Driven, Positive-Sequence)"/2
  "Power (PLL-Driven, Positive-Sequence)"/1 -> PQ->pu/1
  Second-Order Filter2/1 -> P_meas/1
  PQ->pu1/1 -> Second-Order Filter3/1
  Second-Order Filter3/1 -> Q_meas/1
  PQ->pu/1 -> Second-Order Filter2/1
  "Power (PLL-Driven, Positive-Sequence)"/2 -> PQ->pu1/1
  wt/1 -> [wt]
  Saturation/1 -> "Power (PLL-Driven, Positive-Sequence)"/1

== system ts_b04_grid_PASS/Inverter 3 200 kW/Control System/Voltage Regulators ==
  note: Iqref limit set 0.5 pu
  Vq : Inport  PortDimensions=1
  Vq_ref : Inport  Port=2  PortDimensions=1
  On : Inport  Port=3  PortDimensions=1
  Vd : Inport  Port=4  PortDimensions=1
  Vd_ref : Inport  Port=5  PortDimensions=1
  Constant1 : Constant  Value=0
  Constant2 : Constant
  Mux : Mux  Inputs=2
  PI regulator with anti-windup 1 : Subsystem  DialogController=POWERSYS.PowerSysDialog  mask(Discrete PI Controller){Kp=Kp_Vreg, Ki=Ki_Vreg, Par_Limits=[0.5, -0.5], Init=0, Ts=Ts}
      mask prompts: Kp "Proportional gain (Kp):"; Ki "Integral gain (Ki):"; Par_Limits "Output limits: [ Upper   Lower ]"; Init "Output initial value:"; Ts "Sample time:"
      mask help: This block implements a discrete PI controller.
      mask init:
      | UpperLimit=Par_Limits(1);
      | LowerLimit=Par_Limits(2);
      | power_initmask();
      mask Help: This block is part of a subset of blocks in the Extras library that does not have documentation associated with it, other than the block mask description.
      mask Display: disp('PI');
  PI regulator with anti-windup 2 : Subsystem  DialogController=POWERSYS.PowerSysDialog  mask(Discrete PI Controller){Kp=Kp_Vreg, Ki=Ki_Vreg, Par_Limits=Limits_Vreg, Init=0, Ts=Ts}
      mask prompts: Kp "Proportional gain (Kp):"; Ki "Integral gain (Ki):"; Par_Limits "Output limits: [ Upper   Lower ]"; Init "Output initial value:"; Ts "Sample time:"
      mask help: This block implements a discrete PI controller.
      mask init:
      | UpperLimit=Par_Limits(1);
      | LowerLimit=Par_Limits(2);
      | power_initmask();
      mask Help: This block is part of a subset of blocks in the Extras library that does not have documentation associated with it, other than the block mask description.
      mask Display: disp('PI');
  Sum : Sum  Inputs=|+-
  Sum1 : Sum  Inputs=|+-
  Switch : Switch  Criteria=u2 ~= 0  SaturateOnIntegerOverflow=off  InputSameDT=off
  IdIq_ref : Outport  InitialOutput=0  VectorParamsAs1DForOutWhenUnconnected=off
  wires:
  Constant1/1 -> Switch/1
  On/1 -> Switch/2
  Switch/1 -> PI regulator with anti-windup 2/2(Reset), PI regulator with anti-windup 1/2(Reset)
  Constant2/1 -> Switch/3
  Vq_ref/1 -> Sum/1
  Vq/1 -> Sum/2
  Sum/1 -> PI regulator with anti-windup 1/1(Error)
  Sum1/1 -> PI regulator with anti-windup 2/1(Error)
  Vd/1 -> Sum1/1
  Vd_ref/1 -> Sum1/2
  PI regulator with anti-windup 2/1(Out) -> Mux/2
  Mux/1 -> IdIq_ref/1
  PI regulator with anti-windup 1/1(Out) -> Mux/1

== system ts_b04_grid_PASS/Inverter 3 200 kW/Control System/Vref Generation ==
  note: (Correction for delai of Ts)
  note: (Correction for transformer
      |  D1 connection)
  wt : Inport
  VdVq_conv : Inport  Port=2
  Vdc_meas : Inport  Port=3
  Add1 : Sum  Inputs=++++
  Add2 : Sum
  Complex to Magnitude-Angle : ComplexToMagnitudeAngle
  Constant : Constant  Value=-pi/6
  Constant2 : Constant  Value="[ 0  -2*pi/3  2*pi/3  ]"
  Constant3 : Constant  Value=Vnom_sec*sqrt(2)/sqrt(3)
  Constant4 : Constant  Value=Ts*Fnom*(2*pi)
  Demux1 : Demux  Outputs=2
  Gain1 : Gain  Gain=1/2
  Product : Product  Inputs=*/  RndMeth=Zero
  Product1 : Product  Inputs=*/  RndMeth=Zero
  Product2 : Product  Inputs=**  RndMeth=Zero
  Real-Imag to Complex : RealImagToComplex
  Saturation : Saturate  UpperLimit=1  LowerLimit=0
  Trigonometric Function : Trigonometry
  Vref : Outport  VectorParamsAs1DForOutWhenUnconnected=off
  ModIndex : Outport  Port=2  VectorParamsAs1DForOutWhenUnconnected=off
  wires:
  Constant4/1 -> Add1/4
  wt/1 -> Add1/1
  Product2/1 -> Vref/1
  Trigonometric Function/1 -> Product2/2
  Saturation/1 -> ModIndex/1, Product2/1
  Add2/1 -> Trigonometric Function/1
  Add1/1 -> Add2/2
  Complex to Magnitude-Angle/2 -> Add2/1
  Product/1 -> Product1/2
  Constant3/1 -> Product/2
  Constant/1 -> Add1/3
  Constant2/1 -> Add1/2
  Demux1/2 -> Real-Imag to Complex/2
  Demux1/1 -> Real-Imag to Complex/1
  Real-Imag to Complex/1 -> Complex to Magnitude-Angle/1
  Gain1/1 -> Product/1
  Product1/1 -> Demux1/1
  VdVq_conv/1 -> Product1/1
  Vdc_meas/1 -> Gain1/1
  Complex to Magnitude-Angle/1 -> Saturation/1

== system ts_b04_grid_PASS/Inverter 1 500 kW/Control System/Current Regulator/PI regulator with anti-windup D ==
  note: Anti-windup mechanism: Method of conditionnal integration
      |
      | The integration is suspended if saturation occurs and the
      | control error is of the same sign as the control signal.
      |
      | [1] L.Rundqwist, "Anti-Reset Windup for PID Controllers," Ph.D. Thesis TRFT-1033,
      | Departement of Automatic Control, Lund Institute of Technology, Lund, Sweeden, 1991.
  Error : Inport  SampleTime=Ts
  Compare To Zero : simulink/Logic and Bit Operations/Compare To Zero  relop=>  OutDataTypeStr=uint8  ZeroCross=off
  Compare To Zero1 : simulink/Logic and Bit Operations/Compare To Zero  relop=<  OutDataTypeStr=uint8  ZeroCross=off
  Constant : Constant  Value=0
  Constant1 : Constant  Value=UpperLimit
  Constant3 : Constant  Value=LowerLimit
  Discrete-Time Integrator : DiscreteIntegrator  IntegratorMethod=Integration: Trapezoidal  InitialCondition=Init  SampleTime=Ts  LimitOutput=on  UpperSaturationLimit=UpperLimit  LowerSaturationLimit=LowerLimit  ShowStatePort=on  ICPrevOutput=DiscIntNeverNeededParam  ICPrevScaledInput=DiscIntNeverNeededParam
  Kp4 : Gain  Gain=Kp  SaturateOnIntegerOverflow=on  SampleTime=Ts  OutDataTypeStr=Inherit: Same as input  ParamDataTypeStr=Inherit: Same as input
  Kp5 : Gain  Gain=Ki  SaturateOnIntegerOverflow=on  SampleTime=Ts  OutDataTypeStr=Inherit: Same as input  ParamDataTypeStr=Inherit: Same as input
  Logical Operator : Logic  AllPortsSameDT=off  OutDataTypeStr=boolean
  Logical Operator1 : Logic  AllPortsSameDT=off  OutDataTypeStr=boolean
  Logical Operator2 : Logic  Operator=OR  AllPortsSameDT=off  OutDataTypeStr=boolean
  Relational Operator : RelationalOperator  OutDataTypeStr=boolean  InputSameDT=off
  Relational Operator1 : RelationalOperator  Operator=<=  OutDataTypeStr=boolean  InputSameDT=off
  Saturation2 : Saturate  UpperLimit=UpperLimit  LowerLimit=LowerLimit  SampleTime=Ts
  Sum1 : Sum  InputSameDT=on  SaturateOnIntegerOverflow=on  SampleTime=Ts  OutDataTypeStr=Inherit: Same as first input
  Sum6 : Sum  InputSameDT=on  SaturateOnIntegerOverflow=on  SampleTime=Ts  OutDataTypeStr=Inherit: Same as first input
  Switch : Switch  Criteria=u2 > Threshold  SaturateOnIntegerOverflow=off  InputSameDT=off
  Zero-Order Hold : ZeroOrderHold  SampleTime=Ts
  Out : Outport  SampleTime=Ts  InitialOutput=0  VectorParamsAs1DForOutWhenUnconnected=off
  wires:
  Constant/1 -> Switch/1
  Zero-Order Hold/1 -> Sum1/2, Sum6/1
  Discrete-Time Integrator/State -> Sum1/1
  Sum1/1 -> Relational Operator1/1, Relational Operator/1
  Logical Operator2/1 -> Switch/2
  Relational Operator/1 -> Logical Operator/1  "UpperLimit_is_Reached"
  Relational Operator1/1 -> Logical Operator1/1  "LowerLimit_Is_Reached"
  Constant1/1 -> Relational Operator/2
  Constant3/1 -> Relational Operator1/2
  Compare To Zero/1 -> Logical Operator/2  "Error_is_positive"
  Logical Operator/1 -> Logical Operator2/1
  Logical Operator1/1 -> Logical Operator2/2
  Compare To Zero1/1 -> Logical Operator1/2  "Error_is_negative"
  Error/1 -> Compare To Zero1/1, Compare To Zero/1, Kp4/1, Kp5/1
  Sum6/1 -> Saturation2/1
  Kp4/1 -> Zero-Order Hold/1
  Discrete-Time Integrator/1 -> Sum6/2
  Saturation2/1 -> Out/1
  Switch/1 -> Discrete-Time Integrator/1
  Kp5/1 -> Switch/3

== system ts_b04_grid_PASS/Inverter 1 500 kW/Control System/Voltage Regulators/PI regulator with anti-windup 1 ==
  note: Anti-windup mechanism: Method of conditionnal integration
      |
      | The integration is suspended if saturation occurs and the
      | control error is of the same sign as the control signal.
      |
      | [1] L.Rundqwist, "Anti-Reset Windup for PID Controllers," Ph.D. Thesis TRFT-1033,
      | Departement of Automatic Control, Lund Institute of Technology, Lund, Sweeden, 1991.
  Error : Inport  SampleTime=Ts
  Reset : Inport  Port=2  SampleTime=Ts
  Compare To Zero : simulink/Logic and Bit Operations/Compare To Zero  relop=>  OutDataTypeStr=uint8  ZeroCross=off
  Compare To Zero1 : simulink/Logic and Bit Operations/Compare To Zero  relop=<  OutDataTypeStr=uint8  ZeroCross=off
  Constant : Constant  Value=0
  Constant1 : Constant  Value=UpperLimit
  Constant3 : Constant  Value=LowerLimit
  Discrete-Time Integrator : DiscreteIntegrator  IntegratorMethod=Integration: Trapezoidal  ExternalReset=level  InitialCondition=Init  SampleTime=Ts  LimitOutput=on  UpperSaturationLimit=UpperLimit  LowerSaturationLimit=LowerLimit  ShowStatePort=on  ICPrevOutput=DiscIntNeverNeededParam  ICPrevScaledInput=DiscIntNeverNeededParam
  Kp4 : Gain  Gain=Kp  SaturateOnIntegerOverflow=on  SampleTime=Ts  OutDataTypeStr=Inherit: Same as input  ParamDataTypeStr=Inherit: Same as input
  Kp5 : Gain  Gain=Ki  SaturateOnIntegerOverflow=on  SampleTime=Ts  OutDataTypeStr=Inherit: Same as input  ParamDataTypeStr=Inherit: Same as input
  Logical Operator : Logic  AllPortsSameDT=off  OutDataTypeStr=boolean
  Logical Operator1 : Logic  AllPortsSameDT=off  OutDataTypeStr=boolean
  Logical Operator2 : Logic  Operator=OR  AllPortsSameDT=off  OutDataTypeStr=boolean
  Relational Operator : RelationalOperator  OutDataTypeStr=boolean  InputSameDT=off
  Relational Operator1 : RelationalOperator  Operator=<=  OutDataTypeStr=boolean  InputSameDT=off
  Saturation2 : Saturate  UpperLimit=UpperLimit  LowerLimit=LowerLimit  SampleTime=Ts
  Sum1 : Sum  InputSameDT=on  SaturateOnIntegerOverflow=on  SampleTime=Ts  OutDataTypeStr=Inherit: Same as first input
  Sum6 : Sum  InputSameDT=on  SaturateOnIntegerOverflow=on  SampleTime=Ts  OutDataTypeStr=Inherit: Same as first input
  Switch : Switch  Criteria=u2 > Threshold  SaturateOnIntegerOverflow=off  InputSameDT=off
  Zero-Order Hold : ZeroOrderHold  SampleTime=Ts
  Out : Outport  SampleTime=Ts  InitialOutput=0  VectorParamsAs1DForOutWhenUnconnected=off
  wires:
  Kp5/1 -> Switch/3
  Switch/1 -> Discrete-Time Integrator/1
  Saturation2/1 -> Out/1
  Discrete-Time Integrator/1 -> Sum6/2
  Kp4/1 -> Zero-Order Hold/1
  Sum6/1 -> Saturation2/1
  Error/1 -> Kp5/1, Kp4/1, Compare To Zero/1, Compare To Zero1/1
  Compare To Zero1/1 -> Logical Operator1/2  "Error_is_negative"
  Logical Operator1/1 -> Logical Operator2/2
  Logical Operator/1 -> Logical Operator2/1
  Compare To Zero/1 -> Logical Operator/2  "Error_is_positive"
  Constant3/1 -> Relational Operator1/2
  Constant1/1 -> Relational Operator/2
  Relational Operator1/1 -> Logical Operator1/1  "LowerLimit_Is_Reached"
  Relational Operator/1 -> Logical Operator/1  "UpperLimit_is_Reached"
  Logical Operator2/1 -> Switch/2
  Sum1/1 -> Relational Operator/1, Relational Operator1/1
  Discrete-Time Integrator/State -> Sum1/1
  Zero-Order Hold/1 -> Sum6/1, Sum1/2
  Constant/1 -> Switch/1
  Reset/1 -> Discrete-Time Integrator/2
